simulink model "free_fall_slx"  (R2026a)
settings: Solver=VariableStepAuto  StopTime=10
values from neighbouring files (symbols this model uses):
  c = 100000    [parameters.m]
  d = 30000    [parameters.m]
  g = 9.81    [parameters.m]
  h0 = 0.5    [parameters.m]
  m = 500    [parameters.m]
settings Model: Creator=s2510444032  LastModifiedBy=s2510444032

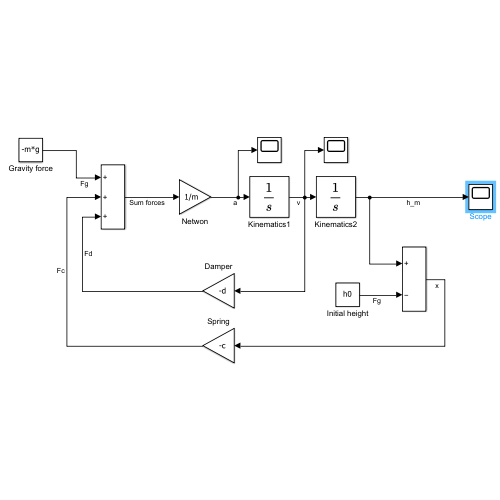
[thumbnail: Simulink's stored preview of the top-level diagram]
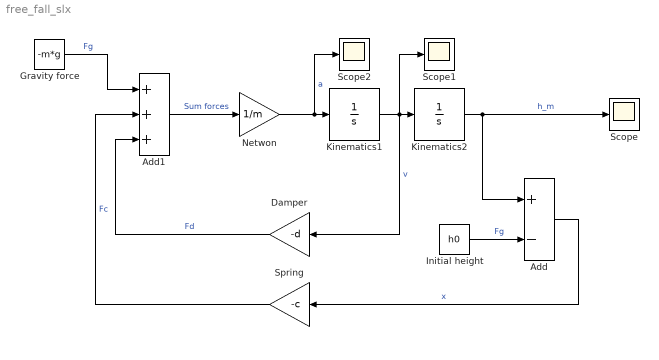
== system free_fall_slx ==
  Add : Sum  Inputs=+-
  Add1 : Sum  Inputs=+++
  Damper : Gain  Gain=-d
  Gravity force : Constant  Value=-m*g
  Initial height : Constant  Value=h0
  Kinematics1 : Integrator
  Kinematics2 : Integrator  InitialCondition=h0
  Netwon : Gain  Gain=1/m
  Scope : Scope
      settings: ActiveDisplayYMinimum=0.40085530592135477  ActiveDisplayYMaximum=0.51101607711984953
  Scope1 : Scope
      settings: ActiveDisplayYMinimum=-5.5181249999999959  ActiveDisplayYMaximum=0.61312499999999948
  Scope2 : Scope
      settings: ActiveDisplayYMinimum=-0.87953124999999877  ActiveDisplayYMaximum=0.65328124999999981  DataLoggingVariableName=ScopeData2
  Spring : Gain  Gain=-c
  wires:
  Netwon/1 -> Scope2/1, Kinematics1/1  "a"
  Kinematics1/1 -> Damper/1, Kinematics2/1, Scope1/1  "v"
  Gravity force/1 -> Add1/1  "Fg"
  Kinematics2/1 -> Add/1, Scope/1  "h_m"
  Initial height/1 -> Add/2  "Fg"
  Add/1 -> Spring/1  "x"
  Spring/1 -> Add1/2  "Fc"
  Add1/1 -> Netwon/1  "Sum forces"
  Damper/1 -> Add1/3  "Fd"
